simulink model "s_b4a4x1kf_nb"  (R2016b)
settings: Solver=VariableStepDiscrete  StartTime=0.0  StopTime=1  RelTol=1e-3
undefined symbols (not defined in the file): fft_stages, n_bits_ants, n_bits_xengs
libraries: xbsIndex_r4 x20504, casper_library_misc x167, casper_library_scopes x13, casper_library_delays x13, xbsReplacements_r4 x6, xps_library x3
(part 23 of 176)

== system s_b4a4x1kf_nb/sys0/snap_xeng_int ==
  in_data : Inport
  in_dv : Inport  Port=2
  in_sync : Inport  Port=3
  in_winvalid : Inport  Port=4
  we : Inport  Port=5
  trig : Inport  Port=6
  assert_data : xbsIndex_r4/Assert  assert_type=on  type_source=Explicitly  gui_display_data_type=Fixed-point  arith_type=Unsigned  n_bits=25  bin_pt=0  preci_type=Single  exp_width=8  frac_width=24  assert_rate=off  rate_source=Explicitly  period=1  output_port=on  block_type=assert
  assert_dv : xbsIndex_r4/Assert  assert_type=on  type_source=Explicitly  gui_display_data_type=Boolean  arith_type=Boolean  n_bits=1  bin_pt=0  preci_type=Single  exp_width=8  frac_width=24  assert_rate=off  rate_source=Explicitly  period=1  output_port=on  block_type=assert
  assert_sync : xbsIndex_r4/Assert  assert_type=on  type_source=Explicitly  gui_display_data_type=Boolean  arith_type=Boolean  n_bits=1  bin_pt=0  preci_type=Single  exp_width=8  frac_width=24  assert_rate=off  rate_source=Explicitly  period=1  output_port=on  block_type=assert
  assert_winvalid : xbsIndex_r4/Assert  assert_type=on  type_source=Explicitly  gui_display_data_type=Boolean  arith_type=Boolean  n_bits=1  bin_pt=0  preci_type=Single  exp_width=8  frac_width=24  assert_rate=off  rate_source=Explicitly  period=1  output_port=on  block_type=assert
  buscreate : Subsystem  AncestorBlock=casper_library_flow_control/bus_create  mask(bus_create){inputNum=4}
      mask prompts: inputNum "Number of inputs:"
      mask init:
      | bus_create_init(gcb,...
      |     'inputNum', inputNum);
  ss : Subsystem  Tag=casper:snapshot  AncestorBlock=casper_library_scopes/snapshot  mask(snapshot){storage=bram, dram_dimm=2, dram_clock=250, nsamples=13, data_width=32, offset=on, circap=off, value=off, ext_arm=off, ext_circ=off, provide_outputs=off, use_dsp48=off}
      mask prompts: storage "Storage medium"; dram_dimm "DRAM dimm"; dram_clock "DRAM clock rate"; nsamples "Number of Samples (2^?)"; data_width "Data width"; offset "Start delay support"; circap "Circular capture support"; value "Extra value capture support"; ext_arm "External arm support"; ext_circ "External circular capture support"; provide_outputs "Provide outputs"; use_dsp48 "Use DSP48s to implement counters"
      mask help:
      | Standard snap block, but with the following optional extras;
      |  1) Optionally delay the fabric trigger by a user-specified number of valids.
      |  2) Capture continuously after a trigger until a stop pulse is received. Data is captured into BRAM continuously, with old data being overwritten until a stop command is received. Then stop capturing when memory is filled. This enables you to get some data before and some data after the stop pulse. Use the 'tr_en_cnt' register to determine where you are in your vector. 'Addr' register's MSb now indicates 'busy capturing'.
      |  3) Optionally capture a value on an input port to a register at the same time as the first data sample.
      |  4) Implement counters using DSP48Es to save resources.
      mask init: same as s_b4a4x1kf_nb/snap_gbe0_rx/ss
      settings: AttributesFormatString=|
      | 32 wide, 8192 deep
      | debugID: 39833321
      mask TypeOptions storage: bram | dram
      mask Callback storage: snapshot_callback();
      mask TypeOptions dram_dimm: 1 | 2 | 3 | 4
      mask TypeOptions dram_clock: 200 | 250 | 266 | 300 | 333
      mask TypeOptions data_width: 8 | 16 | 32 | 64 | 128
  arm_out : Outport
  wires:
  ss/1(arm_out) -> arm_out/1
  buscreate/1(bus_out) -> ss/1(din)
  in_data/1 -> assert_data/1
  assert_data/1 -> buscreate/1(in1)
  in_dv/1 -> assert_dv/1
  assert_dv/1 -> buscreate/2(in2)
  in_sync/1 -> assert_sync/1
  assert_sync/1 -> buscreate/3(in3)
  in_winvalid/1 -> assert_winvalid/1
  assert_winvalid/1 -> buscreate/4(in4)
  we/1 -> ss/2(we)
  trig/1 -> ss/3(trig)

== system s_b4a4x1kf_nb/sys0/vacc ==
  cnt_rst : Inport
  arm : Inport  Port=2
  start_time : Inport  Port=3
  immediate : Inport  Port=4
  acc_len : Inport  Port=5
  data_in : Inport  Port=6
  we : Inport  Port=7
  timestamp_in : Inport  Port=8
  re : Inport  Port=9
  Reinterpret1 : xbsIndex_r4/Reinterpret  force_arith_type=on  arith_type=Unsigned  force_bin_pt=on  bin_pt=0  block_type=reinterpret
      settings: block_version=10.1.3
  Subsystem : Subsystem  mask{cnt_bits=4}
  delay1 : xbsIndex_r4/Delay  rst=off  infoeditControl=Selection of Reset will increase slice count due to use of real FFs and instead of SRLs  en=off  latency=2  reg_retiming=on  dbl_ovrd=off  block_type=delay
  delay{2,6..8,10..12} (7 alike) : xbsIndex_r4/Delay  rst=off  infoeditControl=Selection of Reset will increase slice count due to use of real FFs and instead of SRLs  en=off  latency=1  reg_retiming=on  dbl_ovrd=off  block_type=delay
      settings: infoedit=Hardware notes: A delay line is a chain, each link of which is an SRL16 or SRL32 followed by a flip-flop.
  delay3 : xbsIndex_r4/Delay  rst=off  infoeditControl=Selection of Reset will increase slice count due to use of real FFs and instead of SRLs  en=off  latency=2  reg_retiming=on  dbl_ovrd=off  block_type=delay
  edge_detect4 : casper_library_misc/edge_detect  edge=Rising  polarity=Active High  x_in=[0 0.08 0.08 0.16 0.16 0.24 0.24 0.32 0.32 0.4]  y_in="[-1 -1  1  1  1  1  1  1  1  1]"  x_out=[0.6 0.68 0.68 0.76 0.76 0.84 0.84 0.92 0.92 1]  y_out="[-1 -1  1  1 -1 -1 -1 -1 -1 -1]"
  hmc_vacc : Subsystem  mask{vector_len=vector_len, mezz=0, n_bits=n_bits, n_inputs=n_inputs}
      mask prompts: vector_len "Vector length??(# cycles)"; mezz "Which HMC Mezzanine slot?"; n_bits "Data width (bits)"; n_inputs "Simultaneous inputs (2^?)"
      mask help:
      | A vector accumulator for medium length vectors designed for ROACH's QDR memory.
      |
      | Originally designed for the packetised correlator, this block accepts input data of type Fix_32_0. OOB_data_in provides an extra 4 bits that are accumulated seperately (originally designed to keep track of how many "bad" values in a vector were accumulated).
      |
      | Minimum vector length is 2 * burst_length.
      | Minimum burst length is 10 (recommended default is 2^4=16).
      |
      | The vector length does not need to be a multiple of the burst length.
      mask init:
      | vector_bits = ceil(log2(vector_len));
      | set_param([gcb, '/hmc'], 'mez', mezz);
      | 
      | fmtstr = sprintf('Vector Length: %d', vector_len);
      | set_param(gcb, 'AttributesFormatString', fmtstr);
      settings: AttributesFormatString=Vector Length: 2560
      mask TypeOptions mezz: 0 | 1 | 2 | 3
  pipeline : Subsystem  AncestorBlock=casper_library_delays/pipeline  mask(pipeline){latency=1}
      mask help:
      | An explicitly laid-out delay line to avoid mapping to SRL16s
      | for use in pipelining to help achieve timing closure.
      mask init:
      | pipeline_init(gcb,'latency',latency);
      settings: AttributesFormatString=Latency = %<latency>
      mask Display:
      | port_label('input', 1, 'd');
      | port_label('output', 1, 'q');
      | disp(['Z^-', num2str(latency)]);
  status : Subsystem  Tag=xps:sw_reg  AncestorBlock=xps_library/software register  mask(swreg){io_dir=To Processor, io_delay=1, sample_period=1, names=[acc_cnt err_cnt arm_cnt ld_cnt], bitwidths=[12 12 4 4], bin_pts=0, arith_types=0, sim_port=off, show_format=off}
      mask prompts: io_dir "I/O direction"; io_delay "I/O delay"; sample_period "Sample period"; names "Bitfield names [msb...lsb]"; bitwidths "Bitfield widths"; bin_pts "Bitfield binary pts"; arith_types "Bitfield types, ufix=0, fix=1, bool=2"; sim_port "Provide sim input/output?"; show_format "Print format string?"
      mask help: A 32-bit software-accessible register. Can be divided into bitfields of varying widths and types using the fields in the block mask.
      mask init:
      | try
      |     swreg_init(gcb)
      | catch ex
      |     disp(sprintf('%s: %s', gcb, ex.message))
      |     errordlg(ex.message)
      | end
      settings: AttributesFormatString=4 outputs
      mask TypeOptions io_dir: To Processor | From Processor
      mask Callback io_dir:
      | mask_enables = get_param(gcb, 'MaskEnables');
      | mask_names = get_param(gcb, 'MaskNames');
      | if strcmp(get_param(gcb, 'io_dir'), 'To Processor'),
      |     mask_enables{ismember(mask_names, 'sample_period')} = 'off';
      | else
      |     mask_enables{ismember(mask_names, 'sample_period')} = 'on';
      | end
      | set_param(gcb, 'MaskEnables', mask_enables);
  time_latch : xbsIndex_r4/Register  init=0  rst=off  en=on  dbl_ovrd=off  block_type=register
  timestamp : Subsystem  Tag=xps:sw_reg  AncestorBlock=xps_library/software_register  mask(swreg){io_dir=To Processor, io_delay=0, sample_period=1, names=vacc_timestamp, bitwidths=26, bin_pts=0, arith_types=0, sim_port=off, show_format=on}
      mask prompts: io_dir "I/O direction"; io_delay "I/O delay"; sample_period "Sample period"; names "Bitfield names [msb...lsb]"; bitwidths "Bitfield widths"; bin_pts "Bitfield binary pts"; arith_types "Bitfield types, ufix=0, fix=1, bool=2"; sim_port "Provide sim input/output?"; show_format "Print format string?"
      mask help: A 32-bit software-accessible register. Can be divided into bitfields of varying widths and types using the fields in the block mask.
      mask init:
      | swreg_init(gcb)
      settings: AttributesFormatString=1output:uf26.0 = 26 bits
      mask TypeOptions io_dir: To Processor | From Processor
      mask Callback io_dir:
      | mask_enables = get_param(gcb, 'MaskEnables');
      | mask_names = get_param(gcb, 'MaskNames');
      | if strcmp(get_param(gcb, 'io_dir'), 'To Processor'),
      |     mask_enables{ismember(mask_names, 'sample_period')} = 'off';
      | else
      |     mask_enables{ismember(mask_names, 'sample_period')} = 'on';
      | end
      | set_param(gcb, 'MaskEnables', mask_enables);
      mask DialogControl ParameterTabVar0 Prompt: Setup
  vacc_monitor1 : Subsystem
  vacc_time : Subsystem
  data_out : Outport
  valid_out : Outport  Port=2
  rb_done : Outport  Port=3
  timestamp_out : Outport  Port=4
  error_out : Outport  Port=5
  pkt_rdy : Outport  Port=6
  wires:
  start_time/1 -> delay11/1
  hmc_vacc/4(RB_done) -> [rb_done], rb_done/1
  we/1 -> time_latch/2, delay6/1
  hmc_vacc/3(error) -> [err], error_out/1
  data_in/1 -> delay7/1
  acc_len/1 -> delay8/1
  arm/1 -> delay10/1
  Reinterpret1/1 -> delay3/1
  delay7/1 -> Reinterpret1/1
  delay6/1 -> vacc_time/3(valid_in), delay1/1
  timestamp_in/1 -> time_latch/1
  immediate/1 -> delay12/1
  [rb_done] -> vacc_time/4(rb_done)
  time_latch/1 -> vacc_time/1(timestamp_in)
  delay8/1 -> vacc_time/2(acc_len), hmc_vacc/2(n_acum)
  edge_detect4/1 -> vacc_monitor1/2(new_acc)
  [err] -> vacc_monitor1/3(error)
  vacc_monitor1/1(acc_cnt) -> status/1(out_acc_cnt)
  vacc_monitor1/2(error_cnt) -> status/2(out_err_cnt)
  [rb_done] -> edge_detect4/1
  vacc_time/1(timestamp_out) -> timestamp_out/1, pipeline/1(d)
  pipeline/1(q) -> timestamp/1(out_vacc_timestamp)
  Subsystem/1(arm_count) -> status/3(out_arm_cnt)
  Subsystem/2(ld_count) -> status/4(out_ld_cnt)
  cnt_rst/1 -> delay2/1
  [vacc_armed] -> Subsystem/2(armed)
  vacc_time/2(armed) -> [vacc_armed]
  delay2/1 -> Subsystem/1(cnt_rst1), vacc_monitor1/1(cnt_rst)
  delay10/1 -> vacc_time/5(arm)
  delay11/1 -> vacc_time/6(load_time)
  delay12/1 -> vacc_time/7(immediate)
  hmc_vacc/1(data_out) -> data_out/1
  hmc_vacc/2(valid) -> valid_out/1
  hmc_vacc/5(pkt_rdy) -> pkt_rdy/1
  delay1/1 -> hmc_vacc/4(valid_data)
  [vacc_armed] -> hmc_vacc/1(rst)
  delay3/1 -> hmc_vacc/3(data_in)
  re/1 -> hmc_vacc/5(ack_RB)

== system s_b4a4x1kf_nb/sys0/vacc_tvg0 ==
  note: This counter increments by
      | one per accumulation.
      | Might be buggy; not tested.
  note: this TVG injects the same
      | number for vector_len.
      | Increments on vector edge.
      | (ramp over time)
  note: this TVG increments on
      | each valid input and resets
      | on vector_edge.
      | (ramp over channels).
  sync_in : Inport
  valid_in : Inport  Port=2
  data_in : Inport  Port=3
  time_in : Inport  Port=4
  acc_start_time : Inport  Port=5
  acc_len : Inport  Port=6
  Delay{,2..8} (8 alike) : xbsIndex_r4/Delay  rst=off  infoeditControl=Selection of Reset will increase slice count due to use of real FFs and instead of SRLs  en=off  latency=1  reg_retiming=on  dbl_ovrd=off  block_type=delay
      Delay settings: xl_area=[0, 0, 0, 0, 0, 0, 0]
      Delay2 settings: infoedit=Hardware notes: A delay line is a chain, each link of which is an SRL16 or SRL32 followed by a flip-flop.  xl_area=[0, 0, 0, 0, 0, 0, 0]
  Delay1 : xbsIndex_r4/Delay  rst=off  infoeditControl=Selection of Reset will increase slice count due to use of real FFs and instead of SRLs  en=off  latency=2  reg_retiming=on  dbl_ovrd=off  block_type=delay
      settings: infoedit=Hardware notes: A delay line is a chain, each link of which is an SRL16 or SRL32 followed by a flip-flop.  xl_area=[0, 0, 0, 0, 0, 0, 0]
  Delay9 : xbsIndex_r4/Delay  rst=off  infoeditControl=Selection of Reset will increase slice count due to use of real FFs and instead of SRLs  en=off  latency=3  reg_retiming=on  dbl_ovrd=off  block_type=delay
      settings: infoedit=Hardware notes: A delay line is a chain, each link of which is an SRL16 or SRL32 followed by a flip-flop.
  Mux1 : xbsIndex_r4/Mux  inputs=2  en=off  latency=1  precision=Full  arith_type="Signed  (2's comp)"  n_bits=8  bin_pt=2  quantization=Truncate  overflow=Wrap  dbl_ovrd=off  block_type=mux
      settings: xl_area=[0, 0, 0, 0, 0, 0, 0]
  Mux2 : xbsIndex_r4/Mux  inputs=2  en=off  latency=1  precision=Full  arith_type="Signed  (2's comp)"  n_bits=8  bin_pt=2  quantization=Truncate  overflow=Wrap  dbl_ovrd=off  block_type=mux
      settings: xl_area=[0, 0, 0, 0, 0, 0, 0]
  Mux3 : xbsIndex_r4/Mux  inputs=2  en=off  latency=1  precision=Full  arith_type="Signed  (2's comp)"  n_bits=8  bin_pt=2  quantization=Truncate  overflow=Wrap  dbl_ovrd=off  block_type=mux
      settings: xl_area=[0, 0, 0, 0, 0, 0, 0]
  Pulse Generator3 : DiscretePulseGenerator  Amplitude=25  Period=99999999  PulseWidth=500000  PhaseDelay=450000
  Relational2 : xbsIndex_r4/Relational  mode=a=b  op_type=Bool  en=off  latency=1  dbl_ovrd=off  block_type=relational
      settings: block_version=10.1.3
  Slice8 : xbsIndex_r4/Slice  nbits=n_bits  boolean_output=off  mode=Lower Bit Location + Width  bit1=0  base1=MSB of Input  bit0=0  base0=LSB of Input  dbl_ovrd=off  block_type=slice
  Slice9 : xbsIndex_r4/Slice  nbits=n_bits  boolean_output=off  mode=Lower Bit Location + Width  bit1=0  base1=MSB of Input  bit0=0  base0=LSB of Input  dbl_ovrd=off  block_type=slice
  Terminator5 : Terminator
  bus_replicate1 : Subsystem  AncestorBlock=casper_library_bus/bus_replicate  mask(bus_replicate){replication=n_inputs, latency=0, misc=off, implementation=core}
      mask prompts: replication "replication factor"; misc "misc support"; implementation "delay implementation"
      mask help: Output bus formed by replicating input bus a number of times
      mask init:
      | bus_replicate_init(gcb, ...
      |     'replication', replication, ...
      |     'latency', latency, ...
      |     'implementation', implementation, ...
      |     'misc', misc);
      mask TypeOptions implementation: core | behavioral
  bus_replicate2 : Subsystem  AncestorBlock=casper_library_bus/bus_replicate  mask(bus_replicate){replication=n_inputs, latency=0, misc=off, implementation=core}
      mask prompts: replication "replication factor"; misc "misc support"; implementation "delay implementation"
      mask help: Output bus formed by replicating input bus a number of times
      mask init:
      | bus_replicate_init(gcb, ...
      |     'replication', replication, ...
      |     'latency', latency, ...
      |     'implementation', implementation, ...
      |     'misc', misc);
      mask TypeOptions implementation: core | behavioral
  edge_detect : Subsystem  AncestorBlock=casper_library_misc/edge_detect  mask(edge_detect){edge=Rising, polarity=Active High, x_in=[0 0.08 0.08 0.16 0.16 0.24 0.24 0.32 0.32 0.4], y_in=[-1 -1  1  1  1  1  1  1  1  1], x_out=[0.6 0.68 0.68 0.76 0.76 0.84 0.84 0.92 0.92 1], y_out=[-1 -1  1  1 -1 -1 -1 -1 -1 -1]}
      mask prompts: edge "Edge Type"; polarity "Output Polarity"; x_in "Input X Positions"; y_in "Input Y Positions"; x_out "Output X Positions"; y_out "Output Y Positions"
      mask help: Output is active for one-cycle after each edge of the specified type (i.e. rising, falling or both).
      mask init: same as s_b4a4x1kf_nb/edge_detect
      settings: AttributesFormatString=|
      | rising edges
      | active high
      mask Help: Output is active for one-cycle after each edge of the specified type (i.e. rising, falling, or both).  Latency is zero.
      mask TypeOptions edge: Rising | Falling | Both
      mask TypeOptions polarity: Active High | Active Low
      mask Display:
      | plot(x_in_num,0.5+y_in_num*0.2);
      | plot(x_out_num,0.5+y_out_num*0.2);
  edge_detect4 : Subsystem  AncestorBlock=casper_library_misc/edge_detect  mask(edge_detect){edge=Rising, polarity=Active High, x_in=[0 0.08 0.08 0.16 0.16 0.24 0.24 0.32 0.32 0.4], y_in=[-1 -1  1  1  1  1  1  1  1  1], x_out=[0.6 0.68 0.68 0.76 0.76 0.84 0.84 0.92 0.92 1], y_out=[-1 -1  1  1 -1 -1 -1 -1 -1 -1]}
      mask prompts: edge "Edge Type"; polarity "Output Polarity"; x_in "Input X Positions"; y_in "Input Y Positions"; x_out "Output X Positions"; y_out "Output Y Positions"
      mask help: Output is active for one-cycle after each edge of the specified type (i.e. rising, falling or both).
      mask init: same as s_b4a4x1kf_nb/edge_detect
      settings: AttributesFormatString=|
      | rising edges
      | active high
      mask Help: Output is active for one-cycle after each edge of the specified type (i.e. rising, falling, or both).  Latency is zero.
      mask TypeOptions edge: Rising | Falling | Both
      mask TypeOptions polarity: Active High | Active Low
      mask Display:
      | plot(x_in_num,0.5+y_in_num*0.2);
      | plot(x_out_num,0.5+y_out_num*0.2);
  generate_pulses : Subsystem
  generate_time : Subsystem  mask{vec_len=len, n_inputs=n_inputs, n_bits=n_bits}
      mask prompts: vec_len "Vector Length?"; n_inputs "Simultaneous inputs"; n_bits "Data width"
      mask init:
      | vector_bits=ceil(log2(vec_len));
      | fmtstr = sprintf('Vector Length: %d', vec_len);
      | set_param(gcb, 'AttributesFormatString', fmtstr);
      settings: AttributesFormatString=Vector Length: 2560
  group_period : Subsystem  Tag=xps:sw_reg  AncestorBlock=xps_library/software register  mask(swreg){io_dir=From Processor, io_delay=0, sample_period=1, names=reg, bitwidths=32, bin_pts=0, arith_types=0, sim_port=on, show_format=on}
      mask prompts: io_dir "I/O direction"; io_delay "I/O delay"; sample_period "Sample period"; names "Bitfield names [msb...lsb]"; bitwidths "Bitfield widths"; bin_pts "Bitfield binary pts"; arith_types "Bitfield types, ufix=0, fix=1, bool=2"; sim_port "Provide sim input/output?"; show_format "Print format string?"
      mask help: A 32-bit software-accessible register. Can be divided into bitfields of varying widths and types using the fields in the block mask.
      mask init:
      | swreg_init(gcb)
      settings: AttributesFormatString=1input:uf32.0 = 32 bits
      mask TypeOptions io_dir: To Processor | From Processor
      mask Callback io_dir:
      | mask_enables = get_param(gcb, 'MaskEnables');
      | mask_names = get_param(gcb, 'MaskNames');
      | if strcmp(get_param(gcb, 'io_dir'), 'To Processor'),
      |     mask_enables{ismember(mask_names, 'sample_period')} = 'off';
      | else
      |     mask_enables{ismember(mask_names, 'sample_period')} = 'on';
      | end
      | set_param(gcb, 'MaskEnables', mask_enables);
  ins_counter : Subsystem  mask{vec_len=len, n_inputs=n_inputs, n_bits=n_bits}
      mask prompts: vec_len "Vector Length?"; n_inputs "Simultaneous inputs"; n_bits "Data width"
      mask init:
      | fmtstr = sprintf('Vector Length: %d', vec_len);
      | set_param(gcb, 'AttributesFormatString', fmtstr);
      settings: AttributesFormatString=Vector Length: 2560
  ins_counter2 : Subsystem  mask{vec_len=len, n_inputs=n_inputs, n_bits=n_bits}
      mask prompts: vec_len "Vector Length?"; n_inputs "Simultaneous inputs"; n_bits "Data width"
      mask init:
      | vector_bits=ceil(log2(vec_len));
      | fmtstr = sprintf('Vector Length: %d', vec_len);
      | set_param(gcb, 'AttributesFormatString', fmtstr);
      settings: AttributesFormatString=Vector Length: 2560
  ins_counter3 : Subsystem  mask{vec_len=len, n_inputs=n_inputs, n_bits=n_bits}
      mask prompts: vec_len "Vector Length?"; n_inputs "Simultaneous inputs"; n_bits "Data width"
      mask init:
      | vector_bits=ceil(log2(vec_len));
      | fmtstr = sprintf('Vector Length: %d', vec_len);
      | set_param(gcb, 'AttributesFormatString', fmtstr);
      settings: AttributesFormatString=Vector Length: 2560
  ins_vect_loc : Subsystem  Tag=xps:sw_reg  AncestorBlock=xps_library/software register  mask(swreg){io_dir=From Processor, io_delay=0, sample_period=1, names=reg, bitwidths=32, bin_pts=0, arith_types=0, sim_port=on, show_format=on}
      mask prompts: io_dir "I/O direction"; io_delay "I/O delay"; sample_period "Sample period"; names "Bitfield names [msb...lsb]"; bitwidths "Bitfield widths"; bin_pts "Bitfield binary pts"; arith_types "Bitfield types, ufix=0, fix=1, bool=2"; sim_port "Provide sim input/output?"; show_format "Print format string?"
      mask help: A 32-bit software-accessible register. Can be divided into bitfields of varying widths and types using the fields in the block mask.
      mask init:
      | swreg_init(gcb)
      settings: AttributesFormatString=1input:uf32.0 = 32 bits
      mask TypeOptions io_dir: To Processor | From Processor
      mask Callback io_dir:
      | mask_enables = get_param(gcb, 'MaskEnables');
      | mask_names = get_param(gcb, 'MaskNames');
      | if strcmp(get_param(gcb, 'io_dir'), 'To Processor'),
      |     mask_enables{ismember(mask_names, 'sample_period')} = 'off';
      | else
      |     mask_enables{ismember(mask_names, 'sample_period')} = 'on';
      | end
      | set_param(gcb, 'MaskEnables', mask_enables);
  ins_vect_val : Subsystem  Tag=xps:sw_reg  AncestorBlock=xps_library/software register  mask(swreg){io_dir=From Processor, io_delay=0, sample_period=1, names=reg, bitwidths=32, bin_pts=0, arith_types=0, sim_port=on, show_format=on}
      mask prompts: io_dir "I/O direction"; io_delay "I/O delay"; sample_period "Sample period"; names "Bitfield names [msb...lsb]"; bitwidths "Bitfield widths"; bin_pts "Bitfield binary pts"; arith_types "Bitfield types, ufix=0, fix=1, bool=2"; sim_port "Provide sim input/output?"; show_format "Print format string?"
      mask help: A 32-bit software-accessible register. Can be divided into bitfields of varying widths and types using the fields in the block mask.
      mask init:
      | swreg_init(gcb)
      settings: AttributesFormatString=1input:uf32.0 = 32 bits
      mask TypeOptions io_dir: To Processor | From Processor
      mask Callback io_dir:
      | mask_enables = get_param(gcb, 'MaskEnables');
      | mask_names = get_param(gcb, 'MaskNames');
      | if strcmp(get_param(gcb, 'io_dir'), 'To Processor'),
      |     mask_enables{ismember(mask_names, 'sample_period')} = 'off';
      | else
      |     mask_enables{ismember(mask_names, 'sample_period')} = 'on';
      | end
      | set_param(gcb, 'MaskEnables', mask_enables);
  ins_vector : Subsystem  mask{num_vectors=len}
      mask prompts: num_vectors "number of vectors"
      mask init:
      | fmtstr = sprintf('Vector Length: %d', num_vectors);
      | set_param(gcb, 'AttributesFormatString', fmtstr);
      settings: AttributesFormatString=Vector Length: 2560
  master_reset_sim1 : Constant
  master_reset_sim2 : Constant  Value=51200000
  master_reset_sim3 : Constant  Value=3
  master_reset_sim5 : Constant  Value=7
  master_reset_sim6 : Constant  Value=10
  master_reset_sim7 : Constant
  n_per_group : Subsystem  Tag=xps:sw_reg  AncestorBlock=xps_library/software register  mask(swreg){io_dir=From Processor, io_delay=0, sample_period=1, names=reg, bitwidths=32, bin_pts=0, arith_types=0, sim_port=on, show_format=on}
      mask prompts: io_dir "I/O direction"; io_delay "I/O delay"; sample_period "Sample period"; names "Bitfield names [msb...lsb]"; bitwidths "Bitfield widths"; bin_pts "Bitfield binary pts"; arith_types "Bitfield types, ufix=0, fix=1, bool=2"; sim_port "Provide sim input/output?"; show_format "Print format string?"
      mask help: A 32-bit software-accessible register. Can be divided into bitfields of varying widths and types using the fields in the block mask.
      mask init:
      | swreg_init(gcb)
      settings: AttributesFormatString=1input:uf32.0 = 32 bits
      mask TypeOptions io_dir: To Processor | From Processor
      mask Callback io_dir:
      | mask_enables = get_param(gcb, 'MaskEnables');
      | mask_names = get_param(gcb, 'MaskNames');
      | if strcmp(get_param(gcb, 'io_dir'), 'To Processor'),
      |     mask_enables{ismember(mask_names, 'sample_period')} = 'off';
      | else
      |     mask_enables{ismember(mask_names, 'sample_period')} = 'on';
      | end
      | set_param(gcb, 'MaskEnables', mask_enables);
  n_pulses : Subsystem  Tag=xps:sw_reg  AncestorBlock=xps_library/software register  mask(swreg){io_dir=From Processor, io_delay=0, sample_period=1, names=reg, bitwidths=32, bin_pts=0, arith_types=0, sim_port=on, show_format=on}
      mask prompts: io_dir "I/O direction"; io_delay "I/O delay"; sample_period "Sample period"; names "Bitfield names [msb...lsb]"; bitwidths "Bitfield widths"; bin_pts "Bitfield binary pts"; arith_types "Bitfield types, ufix=0, fix=1, bool=2"; sim_port "Provide sim input/output?"; show_format "Print format string?"
      mask help: A 32-bit software-accessible register. Can be divided into bitfields of varying widths and types using the fields in the block mask.
      mask init:
      | swreg_init(gcb)
      settings: AttributesFormatString=1input:uf32.0 = 32 bits
      mask TypeOptions io_dir: To Processor | From Processor
      mask Callback io_dir:
      | mask_enables = get_param(gcb, 'MaskEnables');
      | mask_names = get_param(gcb, 'MaskNames');
      | if strcmp(get_param(gcb, 'io_dir'), 'To Processor'),
      |     mask_enables{ismember(mask_names, 'sample_period')} = 'off';
      | else
      |     mask_enables{ismember(mask_names, 'sample_period')} = 'on';
      | end
      | set_param(gcb, 'MaskEnables', mask_enables);
  pipeline{1..4,7} (5 alike) : casper_library_delays/pipeline  latency=3
      settings: AttributesFormatString=Latency = %<latency>
  ts_offset : Subsystem  Tag=xps:sw_reg  AncestorBlock=xps_library/software register  mask(swreg){mode=one value, io_dir=From Processor, io_delay=0, sample_period=1, names=reg, bitwidths=32, arith_types=0, bin_pts=0, sim_port=on, show_format=off}
      mask prompts: io_dir "I/O direction"; io_delay "I/O delay"; sample_period "Sample period"; names "Name:"; bitwidths "Bitwidth:"; arith_types "Type (ufix=0, fix=1, bool=2):"; bin_pts "Binary pt:"; sim_port "Provide sim input/output?"; show_format "Print format string?"
      mask init:
      | swreg_init(gcb)
      settings: AttributesFormatString=1input
      mask TypeOptions mode: one value | fields of equal size | fields of arbitrary size
      mask Callback mode: swreg_cb(gcb);
      mask TypeOptions io_dir: To Processor | From Processor
      mask Callback io_dir:
      | mask_enables = get_param(gcb, 'MaskEnables');
      | mask_names = get_param(gcb, 'MaskNames');
      | if strcmp(get_param(gcb, 'io_dir'), 'To Processor'),
      |     mask_enables{ismember(mask_names, 'sample_period')} = 'off';
      | else
      |     mask_enables{ismember(mask_names, 'sample_period')} = 'on';
      | end
      | set_param(gcb, 'MaskEnables', mask_enables);
      mask Callback bitwidths:
      | swreg_maskcheck(gcb);
      | % blk = gcb;
      | % mode = get_param(blk, 'mode');
      | % current_widths = eval(get_param(blk, 'bitwidths'));
      | % if (strcmp(mode, 'one value') || strcmp(mode, 'fields of equal size')) && (length(current_widths) > 1),
      | %     error('Only one width may be specified for this mode.');
      | % elseif strcmp(mode, 'fields of arbitrary size')
      | %     current_names = textscan(strtrim(strrep(strrep(get_param(blk, 'names'), ']', ''), '[', '')), '%s');
      | %     current_names = current_names{1};
      | %     numios = length(current_names);
      | %     if length(current_widths) ~= numios,
      | %         error('%d field names specified, but %d widths?', numios, length(current_widths));
      | %     end
      | % end
      | % total_width = 0;
      | % for ctr = 1 : length(current_widths),
      | %     total_width = total_width + current_widths(ctr);
      | % end
      | % if total_width > 32,
      | %     error('Total width must be 32 or less, set to %d.', total_width);
      | % end
      mask Callback arith_types:
      | [numios, ~, ~, ~, current_types] = swreg_maskcheck(gcb);
      | % blk = gcb;
      | % mode = get_param(blk, 'mode');
      | % current_types = eval(get_param(blk, 'arith_types'));
      | % numios = length(current_types);
      | % if (strcmp(mode, 'one value') || strcmp(mode, 'fields of equal size')) && (length(current_types) > 1),
      | %     error('Only one type may be specified for this mode.');
      | % elseif strcmp(mode, 'fields of arbitrary size')
      | %     current_names = textscan(strtrim(strrep(strrep(get_param(blk, 'names'), ']', ''), '[', '')), '%s');
      | %     current_names = current_names{1};
      | %     numios = length(current_names);
      | %     if length(current_types) ~= numios,
      | %         error('%d field names specified, but %d types?', numios, length(current_types));
      | %     end
      | % end
      | problem = 0;
      | for ctr = 1 : numios,
      |     t = current_types(ctr);
      |     if (t < 0) || (t > 2),
      |         problem = t;
      |         ctr = numios + 1;
      |     end
      | end
      | if problem ~= 0,
      |     error('Type cannot be %i, must be 0, 1 or 2.', problem);
      | end
      mask Callback bin_pts:
      | swreg_maskcheck(gcb);
      | % blk = gcb;
      | % mode = get_param(blk, 'mode');
      | % current_bins = eval(get_param(blk, 'bin_pts'));
      | % if (strcmp(mode, 'one value') || strcmp(mode, 'fields of equal size')) && (length(current_bins) > 1),
      | %     error('Only one binary pt may be specified for this mode.');
      | % elseif strcmp(mode, 'fields of arbitrary size')
      | %     current_names = textscan(strtrim(strrep(strrep(get_param(blk, 'names'), ']', ''), '[', '')), '%s');
      | %     current_names = current_names{1};
      | %     numios = length(current_names);
      | %     if length(current_bins) ~= numios,
      | %         error('%d field names specified, but %d binary pts?', numios, length(current_bins));
      | %     end
      | % end
  write : Subsystem  Tag=xps:sw_reg  AncestorBlock=xps_library/software register  mask(swreg){io_dir=From Processor, io_delay=0, sample_period=1, names=reg, bitwidths=32, bin_pts=0, arith_types=0, sim_port=on, show_format=on}
      mask prompts: io_dir "I/O direction"; io_delay "I/O delay"; sample_period "Sample period"; names "Bitfield names [msb...lsb]"; bitwidths "Bitfield widths"; bin_pts "Bitfield binary pts"; arith_types "Bitfield types, ufix=0, fix=1, bool=2"; sim_port "Provide sim input/output?"; show_format "Print format string?"
      mask help: A 32-bit software-accessible register. Can be divided into bitfields of varying widths and types using the fields in the block mask.
      mask init:
      | swreg_init(gcb)
      settings: AttributesFormatString=1input:uf32.0 = 32 bits
      mask TypeOptions io_dir: To Processor | From Processor
      mask Callback io_dir:
      | mask_enables = get_param(gcb, 'MaskEnables');
      | mask_names = get_param(gcb, 'MaskNames');
      | if strcmp(get_param(gcb, 'io_dir'), 'To Processor'),
      |     mask_enables{ismember(mask_names, 'sample_period')} = 'off';
      | else
      |     mask_enables{ismember(mask_names, 'sample_period')} = 'on';
      | end
      | set_param(gcb, 'MaskEnables', mask_enables);
  data_out : Outport
  valid_out : Outport  Port=2
  time_out : Outport  Port=3
  wires:
  pipeline2/1 -> generate_pulses/4(group period)
  pipeline1/1 -> generate_pulses/3(num_per_group)
  pipeline7/1 -> generate_pulses/2(num_pulses)
  Delay1/1 -> Mux1/3
  write/1(in_reg) -> Slice8/1
  master_reset_sim1/1 -> write/1(sim_1)
  [vacctvg_reset] -> Delay2/1
  valid_in/1 -> Mux1/2
  ins_vector/2(data) -> data_out/1
  ins_vector/3(valid_out) -> valid_out/1
  data_in/1 -> Mux2/2
  sync_in/1 -> Mux3/2
  [vacctvg_sync_sel] -> Mux3/1
  [vacctvg_data_sel] -> Mux2/1
  [vacctvg_valid_sel] -> Mux1/1
  [vacctvg_pulse_en] -> Delay/1
  generate_pulses/1(valid) -> Delay1/1
  edge_detect/1(out) -> Mux3/3
  [vacctvg_vector_en] -> ins_vector/6(enable)
  [vector_loc] -> ins_vector/4(vector)
  [vacctvg_ctr_en] -> ins_counter/4(enable)
  Delay/1 -> generate_pulses/1(run)
  generate_pulses/2(running) -> Terminator5/1
  [vector_val] -> ins_vector/5(value)
  Slice8/1 -> bus_replicate1/1(in)
  bus_replicate1/1(out) -> Mux2/3
  ins_vector/4(misco) -> time_out/1
  n_pulses/1(in_reg) -> pipeline7/1
  n_per_group/1(in_reg) -> pipeline1/1
  group_period/1(in_reg) -> pipeline2/1
  master_reset_sim2/1 -> n_pulses/1(sim_1)
  master_reset_sim3/1 -> n_per_group/1(sim_1)
  master_reset_sim5/1 -> group_period/1(sim_1)
  master_reset_sim7/1 -> ins_vect_loc/1(sim_1)
  master_reset_sim6/1 -> ins_vect_val/1(sim_1)
  ins_vect_loc/1(in_reg) -> pipeline3/1
  ins_vect_val/1(in_reg) -> pipeline4/1
  Slice9/1 -> bus_replicate2/1(in)
  pipeline4/1 -> Slice9/1
  bus_replicate2/1(out) -> [vector_val]
  pipeline3/1 -> [vector_loc]
  Delay2/1 -> edge_detect/1(in)
  ins_counter/1(new_acc_out) -> ins_vector/1(new_acc_in)
  ins_counter/4(misco) -> ins_vector/7(misci)
  ins_counter/2(dout) -> ins_vector/2(data_in)
  ins_counter/3(valid_out) -> ins_vector/3(valid_in)
  ts_offset/1(in_reg) -> Delay8/1
  Pulse Generator3/1 -> ts_offset/1(sim_1)
  ins_counter2/2(dout) -> ins_counter/2(din)
  ins_counter2/3(valid_out) -> ins_counter/3(valid_in)
  ins_counter2/4(time_out) -> ins_counter/5(misci)
  [vacctvg_ctr2_en] -> ins_counter2/4(cnt_tvg_en)
  ins_counter2/1(sync_out) -> ins_counter/1(new_acc_in)
  time_in/1 -> Delay3/1
  Delay8/1 -> generate_time/6(offset)
  [vacctvg_time_sel] -> generate_time/4(time_tvg_en)
  Mux1/1 -> generate_time/3(valid_in)
  Mux2/1 -> generate_time/2(din)
  Mux3/1 -> generate_time/1(sync_in)
  Delay3/1 -> generate_time/5(time_in)
  edge_detect4/1(out) -> Delay9/1, ins_counter3/6(cnt_rst)
  generate_time/1(sync_out) -> Delay7/1
  generate_time/2(dout) -> Delay6/1
  generate_time/3(valid_out) -> Delay5/1
  ins_counter3/1(sync_out) -> ins_counter2/1(sync_in)
  ins_counter3/2(dout) -> ins_counter2/2(din)
  ins_counter3/3(valid_out) -> ins_counter2/3(valid_in)
  ins_counter3/4(time_out) -> ins_counter2/5(time_in)
  [vacctvg_ctr3_en] -> ins_counter3/4(cnt_tvg_en)
  acc_len/1 -> ins_counter3/7(acc_len)
  Relational2/1 -> edge_detect4/1(in)
  acc_start_time/1 -> Relational2/2
  generate_time/4(time_out) -> Relational2/1, Delay4/1
  Delay4/1 -> ins_counter3/5(time_in)
  Delay5/1 -> ins_counter3/3(valid_in)
  Delay6/1 -> ins_counter3/2(din)
  Delay7/1 -> ins_counter3/1(sync_in)
  Delay9/1 -> ins_counter2/6(cnt_rst)

== system s_b4a4x1kf_nb/sys0/valid_bet_sync ==
  sync : Inport
  rst_max : Inport  Port=2
  valid : Inport  Port=3
  Delay14 : xbsIndex_r4/Delay  rst=off  infoeditControl=Selection of Reset will increase slice count due to use of real FFs and instead of SRLs  en=off  latency=1  reg_retiming=on  dbl_ovrd=off  block_type=delay
      settings: xl_area=[0, 0, 0, 0, 0, 0, 0]
  Register3 : xbsIndex_r4/Register  init=0  rst=on  en=on  dbl_ovrd=off  block_type=register
      settings: xl_area=[0, 0, 0, 0, 0, 0, 0]
  Relational5 : xbsIndex_r4/Relational  mode=a>=b  op_type=Bool  en=off  latency=1  dbl_ovrd=off  block_type=relational
      settings: xl_area=[0, 0, 0, 0, 0, 0, 0]  block_version=10.1.3
  valid_cntr : xbsIndex_r4/Counter  cnt_type=Free Running  cnt_to=Inf  operation=Up  start_count=0  cnt_by_val=1  arith_type=Unsigned  n_bits=32  bin_pt=0  load_pin=off  rst=on  en=on  explicit_period=on  period=1  use_behavioral_HDL=off  implementation=Fabric  use_rpm=on  dbl_ovrd=off  block_type=counter
      settings: xl_area=[0, 0, 0, 0, 0, 0, 0]
  warn period Delay140 : xbsReplacements_r4/Warning  period=1
  warn period Register30 : xbsReplacements_r4/Warning  period=1
  warn period Relational50 : xbsReplacements_r4/Warning  period=1
  max_count : Outport
  count : Outport  Port=2
  wires:
  Delay14/1 -> Register3/1
  Relational5/1 -> Register3/3
  Register3/1 -> Relational5/2, max_count/1
  valid_cntr/1 -> Relational5/1, Delay14/1, count/1
  sync/1 -> valid_cntr/1
  rst_max/1 -> Register3/2
  valid/1 -> valid_cntr/2

== system s_b4a4x1kf_nb/sys0/valid_bet_sync1 ==
  sync : Inport
  rst_max : Inport  Port=2
  valid : Inport  Port=3
  Delay14 : xbsIndex_r4/Delay  rst=off  infoeditControl=Selection of Reset will increase slice count due to use of real FFs and instead of SRLs  en=off  latency=1  reg_retiming=on  dbl_ovrd=off  block_type=delay
      settings: xl_area=[0, 0, 0, 0, 0, 0, 0]
  Register3 : xbsIndex_r4/Register  init=0  rst=on  en=on  dbl_ovrd=off  block_type=register
      settings: xl_area=[0, 0, 0, 0, 0, 0, 0]
  Relational5 : xbsIndex_r4/Relational  mode=a>=b  op_type=Bool  en=off  latency=1  dbl_ovrd=off  block_type=relational
      settings: xl_area=[0, 0, 0, 0, 0, 0, 0]  block_version=10.1.3
  valid_cntr : xbsIndex_r4/Counter  cnt_type=Free Running  cnt_to=Inf  operation=Up  start_count=0  cnt_by_val=1  arith_type=Unsigned  n_bits=32  bin_pt=0  load_pin=off  rst=on  en=on  explicit_period=on  period=1  use_behavioral_HDL=off  implementation=Fabric  use_rpm=on  dbl_ovrd=off  block_type=counter
      settings: xl_area=[0, 0, 0, 0, 0, 0, 0]
  warn period Delay140 : xbsReplacements_r4/Warning  period=1
  warn period Register30 : xbsReplacements_r4/Warning  period=1
  warn period Relational50 : xbsReplacements_r4/Warning  period=1
  max_count : Outport
  count : Outport  Port=2
  wires:
  valid/1 -> valid_cntr/2
  rst_max/1 -> Register3/2
  sync/1 -> valid_cntr/1
  valid_cntr/1 -> count/1, Delay14/1, Relational5/1
  Register3/1 -> max_count/1, Relational5/2
  Relational5/1 -> Register3/3
  Delay14/1 -> Register3/1

== system s_b4a4x1kf_nb/sys0/vbs_reord ==
  out_reg : Inport
  assert_reg : xbsIndex_r4/Assert  assert_type=on  type_source=Explicitly  gui_display_data_type=Fixed-point  arith_type=Unsigned  n_bits=32  bin_pt=0  preci_type=Single  exp_width=8  frac_width=24  assert_rate=off  rate_source=Explicitly  period=1  output_port=on  block_type=assert
  cast_gw : xbsIndex_r4/Convert  gui_display_data_type=Fixed-point  arith_type=Unsigned  n_bits=32  bin_pt=0  float_type=Single  exp_bits=8  fraction_bits=24  quantization=Truncate  overflow=Wrap  en=off  latency=1  pipeline=off  dbl_ovrd=off  block_type=convert
  io_delay : xbsIndex_r4/Delay  rst=off  infoeditControl=Selection of Reset will increase slice count due to use of real FFs and instead of SRLs  en=off  latency=0  reg_retiming=on  dbl_ovrd=off  block_type=delay
      settings: infoedit=Hardware notes: A delay line is a chain, each link of which is an SRL16 or SRL32 followed by a flip-flop.
  reint1 : xbsIndex_r4/Reinterpret  force_arith_type=on  arith_type=Unsigned  force_bin_pt=on  bin_pt=0  block_type=reinterpret
  s_b4a4x1kf_nb_sys0_vbs_reord_user_data_in : xbsIndex_r4/Gateway Out  inherit_from_input=off  hdl_port=on  rows=1  columns=1  UseAsDAC=off  DACChannel='1'  interface=None  automatic_assignment=on  address_offset=hex2dec('00')  intf_name=''  intf_description=''  timing_constraint=None  locs_specified=off  LOCs={}  io_standard={}  block_type=gatewayout
  sim_out : Outport
  wires:
  io_delay/1 -> cast_gw/1
  cast_gw/1 -> s_b4a4x1kf_nb_sys0_vbs_reord_user_data_in/1
  s_b4a4x1kf_nb_sys0_vbs_reord_user_data_in/1 -> sim_out/1
  out_reg/1 -> assert_reg/1
  assert_reg/1 -> reint1/1
  reint1/1 -> io_delay/1

== system s_b4a4x1kf_nb/sys0/vbs_xeng ==
  out_reg : Inport
  assert_reg : xbsIndex_r4/Assert  assert_type=on  type_source=Explicitly  gui_display_data_type=Fixed-point  arith_type=Unsigned  n_bits=32  bin_pt=0  preci_type=Single  exp_width=8  frac_width=24  assert_rate=off  rate_source=Explicitly  period=1  output_port=on  block_type=assert
  cast_gw : xbsIndex_r4/Convert  gui_display_data_type=Fixed-point  arith_type=Unsigned  n_bits=32  bin_pt=0  float_type=Single  exp_bits=8  fraction_bits=24  quantization=Truncate  overflow=Wrap  en=off  latency=1  pipeline=off  dbl_ovrd=off  block_type=convert
  io_delay : xbsIndex_r4/Delay  rst=off  infoeditControl=Selection of Reset will increase slice count due to use of real FFs and instead of SRLs  en=off  latency=0  reg_retiming=on  dbl_ovrd=off  block_type=delay
      settings: infoedit=Hardware notes: A delay line is a chain, each link of which is an SRL16 or SRL32 followed by a flip-flop.
  reint1 : xbsIndex_r4/Reinterpret  force_arith_type=on  arith_type=Unsigned  force_bin_pt=on  bin_pt=0  block_type=reinterpret
  s_b4a4x1kf_nb_sys0_vbs_xeng_user_data_in : xbsIndex_r4/Gateway Out  inherit_from_input=off  hdl_port=on  rows=1  columns=1  UseAsDAC=off  DACChannel='1'  interface=None  automatic_assignment=on  address_offset=hex2dec('00')  intf_name=''  intf_description=''  timing_constraint=None  locs_specified=off  LOCs={}  io_standard={}  block_type=gatewayout
  sim_out : Outport
  wires:
  io_delay/1 -> cast_gw/1
  cast_gw/1 -> s_b4a4x1kf_nb_sys0_vbs_xeng_user_data_in/1
  s_b4a4x1kf_nb_sys0_vbs_xeng_user_data_in/1 -> sim_out/1
  out_reg/1 -> assert_reg/1
  assert_reg/1 -> reint1/1
  reint1/1 -> io_delay/1

== system s_b4a4x1kf_nb/sys0/x_cast ==
  in : Inport
  Concat : xbsIndex_r4/Concat  num_inputs=8  dbl_ovrd=off  block_type=concat
      settings: block_version=9.2.01
  Convert{,1..7} (8 alike) : xbsIndex_r4/Convert  gui_display_data_type=Fixed-point  arith_type="Signed  (2's comp)"  n_bits=n_bits_out  bin_pt=fix_pnt_pos  float_type=Single  exp_bits=8  fraction_bits=24  quantization=Truncate  overflow=Wrap  en=off  latency=0  pipeline=off  dbl_ovrd=off  block_type=convert
      settings: block_version=10.1.3
  Slice : xbsIndex_r4/Slice  nbits=n_bits_in  boolean_output=off  mode=Lower Bit Location + Width  bit1=0  base1=MSB of Input  bit0=bit_offsets(1)*n_bits_in  base0=LSB of Input  dbl_ovrd=off  block_type=slice
      settings: infoedit="Extracts a given range of bits from each input sample and presents it at the output.  The output type is ordinarily unsigned with binary point at zero, but can be Boolean when the slice is one bit wide.<P><P>Hardware notes: In hardware this block costs nothing."  block_version=10.1.3
  Slice1 : xbsIndex_r4/Slice  nbits=n_bits_in  boolean_output=off  mode=Lower Bit Location + Width  bit1=0  base1=MSB of Input  bit0=bit_offsets(2)*n_bits_in  base0=LSB of Input  dbl_ovrd=off  block_type=slice
      settings: infoedit="Extracts a given range of bits from each input sample and presents it at the output.  The output type is ordinarily unsigned with binary point at zero, but can be Boolean when the slice is one bit wide.<P><P>Hardware notes: In hardware this block costs nothing."  block_version=10.1.3
  Slice2 : xbsIndex_r4/Slice  nbits=n_bits_in  boolean_output=off  mode=Lower Bit Location + Width  bit1=0  base1=MSB of Input  bit0=bit_offsets(3)*n_bits_in  base0=LSB of Input  dbl_ovrd=off  block_type=slice
      settings: infoedit="Extracts a given range of bits from each input sample and presents it at the output.  The output type is ordinarily unsigned with binary point at zero, but can be Boolean when the slice is one bit wide.<P><P>Hardware notes: In hardware this block costs nothing."  block_version=10.1.3
  Slice3 : xbsIndex_r4/Slice  nbits=n_bits_in  boolean_output=off  mode=Lower Bit Location + Width  bit1=0  base1=MSB of Input  bit0=bit_offsets(4)*n_bits_in  base0=LSB of Input  dbl_ovrd=off  block_type=slice
      settings: infoedit="Extracts a given range of bits from each input sample and presents it at the output.  The output type is ordinarily unsigned with binary point at zero, but can be Boolean when the slice is one bit wide.<P><P>Hardware notes: In hardware this block costs nothing."  block_version=10.1.3
  Slice4 : xbsIndex_r4/Slice  nbits=n_bits_in  boolean_output=off  mode=Lower Bit Location + Width  bit1=0  base1=MSB of Input  bit0=bit_offsets(5)*n_bits_in  base0=LSB of Input  dbl_ovrd=off  block_type=slice
      settings: infoedit="Extracts a given range of bits from each input sample and presents it at the output.  The output type is ordinarily unsigned with binary point at zero, but can be Boolean when the slice is one bit wide.<P><P>Hardware notes: In hardware this block costs nothing."  block_version=10.1.3
  Slice5 : xbsIndex_r4/Slice  nbits=n_bits_in  boolean_output=off  mode=Lower Bit Location + Width  bit1=0  base1=MSB of Input  bit0=bit_offsets(6)*n_bits_in  base0=LSB of Input  dbl_ovrd=off  block_type=slice
      settings: infoedit="Extracts a given range of bits from each input sample and presents it at the output.  The output type is ordinarily unsigned with binary point at zero, but can be Boolean when the slice is one bit wide.<P><P>Hardware notes: In hardware this block costs nothing."  block_version=10.1.3
  Slice6 : xbsIndex_r4/Slice  nbits=n_bits_in  boolean_output=off  mode=Lower Bit Location + Width  bit1=0  base1=MSB of Input  bit0=bit_offsets(7)*n_bits_in  base0=LSB of Input  dbl_ovrd=off  block_type=slice
      settings: infoedit="Extracts a given range of bits from each input sample and presents it at the output.  The output type is ordinarily unsigned with binary point at zero, but can be Boolean when the slice is one bit wide.<P><P>Hardware notes: In hardware this block costs nothing."  block_version=10.1.3
  Slice7 : xbsIndex_r4/Slice  nbits=n_bits_in  boolean_output=off  mode=Lower Bit Location + Width  bit1=0  base1=MSB of Input  bit0=bit_offsets(8)*n_bits_in  base0=LSB of Input  dbl_ovrd=off  block_type=slice
      settings: infoedit="Extracts a given range of bits from each input sample and presents it at the output.  The output type is ordinarily unsigned with binary point at zero, but can be Boolean when the slice is one bit wide.<P><P>Hardware notes: In hardware this block costs nothing."  block_version=10.1.3
  force_re{,1,4,6,8,10,12,14} (8 alike) : xbsIndex_r4/Reinterpret  force_arith_type=on  arith_type="Signed  (2's comp)"  force_bin_pt=on  bin_pt=fix_pnt_pos  block_type=reinterpret
      settings: infoedit="Changes signal type without altering the binary representation.   You can changed the signal between signed and unsigned, and relocate the binary point.<P><P>Hardware notes: In hardware this block costs nothing.<P><P>Example:  Suppose the input is 6 bits wide, signed, with 2 fractional bits, and the output is forced to unsigned with 0 fractional bits.  Then an input of -2.0 (1110.00 in binary 2's complement) becomes an output of 56 (111000 in binary)."  block_version=9.1.01
  force_re{2..3,5,7,9,11,13,15} (8 alike) : xbsIndex_r4/Reinterpret  force_arith_type=on  arith_type=Unsigned  force_bin_pt=on  bin_pt=0  block_type=reinterpret
      settings: infoedit="Changes signal type without altering the binary representation.   You can changed the signal between signed and unsigned, and relocate the binary point.<P><P>Hardware notes: In hardware this block costs nothing.<P><P>Example:  Suppose the input is 6 bits wide, signed, with 2 fractional bits, and the output is forced to unsigned with 0 fractional bits.  Then an input of -2.0 (1110.00 in binary 2's complement) becomes an output of 56 (111000 in binary)."  block_version=9.1.01
  out : Outport
  wires:
  force_re2/1 -> Concat/1
  Convert/1 -> force_re2/1
  Convert1/1 -> force_re3/1
  force_re/1 -> Convert/1
  force_re1/1 -> Convert1/1
  Slice/1 -> force_re/1
  in/1 -> Slice/1, Slice6/1, Slice7/1, Slice5/1, Slice4/1, Slice3/1, Slice2/1, Slice1/1
  Concat/1 -> out/1
  Slice1/1 -> force_re1/1
  force_re3/1 -> Concat/2
  Convert2/1 -> force_re5/1
  force_re4/1 -> Convert2/1
  Slice2/1 -> force_re4/1
  Convert3/1 -> force_re7/1
  force_re6/1 -> Convert3/1
  Slice3/1 -> force_re6/1
  Convert4/1 -> force_re9/1
  force_re8/1 -> Convert4/1
  Slice4/1 -> force_re8/1
  Convert5/1 -> force_re11/1
  force_re10/1 -> Convert5/1
  Slice5/1 -> force_re10/1
  Convert6/1 -> force_re13/1
  force_re12/1 -> Convert6/1
  Slice6/1 -> force_re12/1
  Convert7/1 -> force_re15/1
  force_re14/1 -> Convert7/1
  Slice7/1 -> force_re14/1
  force_re5/1 -> Concat/3
  force_re7/1 -> Concat/4
  force_re9/1 -> Concat/5
  force_re11/1 -> Concat/6
  force_re13/1 -> Concat/7
  force_re15/1 -> Concat/8
